simulink model "Fourteen_bus_simscape_V1o1"  (R2026a)
settings: Solver=ode23t  StopTime=12  FixedStep=0.2  RelTol=1e-2  AbsTol=1e-2  EnableMultiTasking=on
libraries: ee_lib x92, nesl_utility x64, fl_lib x25, eeRmsMeasurement x18, slpidlib x5, eeSmGovernor x2, elec_conv_HighZElecRef x1
(part 2 of 3)

== system Fourteen_bus_simscape_V1o1/Bus 7  ==
  Current and Voltage Sensor (Three-Phase) : ee_lib/Sensors & Transducers/Current and Voltage Sensor (Three-Phase)  port_option=ee.enum.threePhasePort.expanded  vMeasurementType=ee.enum.vmeasurement.ll  outputUnit=ee.enum.unit.si  SRated=100000000 V*A  VRated=0.95 V  I_specify=off  I_priority=None  I=[ 0 0 0 ] A  I_nominal_specify=off  I_nominal_value=1  I_nominal_unit=A  V_specify=off  V_priority=None  V=[ 0 0 0 ] V  V_nominal_specify=off  V_nominal_value=1  V_nominal_unit=V
  Demux : Demux  Outputs=3
  PS-Simulink Converter : nesl_utility/PS-Simulink Converter  PhysicalDomain=network_engine_domain  SubClassName=ps_output  LeftPortType=input  RightPortType=output  PseudoPeriodic=off  Frequencies=[]  VectorFormat=1-D array  Unit=1  AffineConversion=off
  PS-Simulink Converter1 : nesl_utility/PS-Simulink Converter  PhysicalDomain=network_engine_domain  SubClassName=ps_output  LeftPortType=input  RightPortType=output  PseudoPeriodic=off  Frequencies=[]  VectorFormat=1-D array  Unit=1  AffineConversion=off
  RMS Measurement : eeRmsMeasurement/RMS Measurement  LabelModeActiveChoice=Total  F=60  SpecifyHarmonics=off  K=[0 1 2]  Ts=0
      settings: LibrarySourceBlock=|
      | ee_sl_lib/Measurements/RMS
      | Measurement
  A : PMIOPort  Side=Left
  B : PMIOPort  Port=2  Side=Left
  C : PMIOPort  Port=3  Side=Left
  a : PMIOPort  Port=4  Side=Right
  b : PMIOPort  Port=5  Side=Right
  c : PMIOPort  Port=6  Side=Right
  Vabc : Outport  VectorParamsAs1DForOutWhenUnconnected=off
  Iabc : Outport  Port=2  VectorParamsAs1DForOutWhenUnconnected=off
  wires:
  PS-Simulink Converter1/1 -> Iabc/1
  Demux/2 -> RMS Measurement/1
  PS-Simulink Converter/1 -> Demux/1
  RMS Measurement/1 -> Vabc/1
  connections:
  Current and Voltage Sensor (Three-Phase)/RConn1 -- PS-Simulink Converter/LConn1
  Current and Voltage Sensor (Three-Phase)/RConn2 -- PS-Simulink Converter1/LConn1
  Current and Voltage Sensor (Three-Phase)/RConn5 -- c/RConn1
  Current and Voltage Sensor (Three-Phase)/RConn4 -- b/RConn1
  Current and Voltage Sensor (Three-Phase)/RConn3 -- a/RConn1
  Current and Voltage Sensor (Three-Phase)/LConn3 -- C/RConn1
  Current and Voltage Sensor (Three-Phase)/LConn1 -- A/RConn1
  Current and Voltage Sensor (Three-Phase)/LConn2 -- B/RConn1

== system Fourteen_bus_simscape_V1o1/Bus 8  ==
  Current and Voltage Sensor (Three-Phase) : ee_lib/Sensors & Transducers/Current and Voltage Sensor (Three-Phase)  port_option=ee.enum.threePhasePort.expanded  vMeasurementType=ee.enum.vmeasurement.ll  outputUnit=ee.enum.unit.si  SRated=100000000 V*A  VRated=1 V  I_specify=off  I_priority=None  I=[ 0 0 0 ] A  I_nominal_specify=off  I_nominal_value=1  I_nominal_unit=A  V_specify=off  V_priority=None  V=[ 0 0 0 ] V  V_nominal_specify=off  V_nominal_value=1  V_nominal_unit=V
  Demux : Demux  Outputs=3
  PS-Simulink Converter : nesl_utility/PS-Simulink Converter  PhysicalDomain=network_engine_domain  SubClassName=ps_output  LeftPortType=input  RightPortType=output  PseudoPeriodic=off  Frequencies=[]  VectorFormat=1-D array  Unit=1  AffineConversion=off
  PS-Simulink Converter1 : nesl_utility/PS-Simulink Converter  PhysicalDomain=network_engine_domain  SubClassName=ps_output  LeftPortType=input  RightPortType=output  PseudoPeriodic=off  Frequencies=[]  VectorFormat=1-D array  Unit=1  AffineConversion=off
  RMS Measurement : eeRmsMeasurement/RMS Measurement  LabelModeActiveChoice=Total  F=60  SpecifyHarmonics=off  K=[0 1 2]  Ts=0
      settings: LibrarySourceBlock=|
      | ee_sl_lib/Measurements/RMS
      | Measurement
  A : PMIOPort  Side=Left
  B : PMIOPort  Port=2  Side=Left
  C : PMIOPort  Port=3  Side=Left
  a : PMIOPort  Port=4  Side=Right
  b : PMIOPort  Port=5  Side=Right
  c : PMIOPort  Port=6  Side=Right
  Vabc : Outport  VectorParamsAs1DForOutWhenUnconnected=off
  Iabc : Outport  Port=2  VectorParamsAs1DForOutWhenUnconnected=off
  wires:
  PS-Simulink Converter1/1 -> Iabc/1
  Demux/2 -> RMS Measurement/1
  PS-Simulink Converter/1 -> Demux/1
  RMS Measurement/1 -> Vabc/1
  connections:
  Current and Voltage Sensor (Three-Phase)/RConn1 -- PS-Simulink Converter/LConn1
  Current and Voltage Sensor (Three-Phase)/RConn2 -- PS-Simulink Converter1/LConn1
  Current and Voltage Sensor (Three-Phase)/RConn5 -- c/RConn1
  Current and Voltage Sensor (Three-Phase)/RConn4 -- b/RConn1
  Current and Voltage Sensor (Three-Phase)/RConn3 -- a/RConn1
  Current and Voltage Sensor (Three-Phase)/LConn3 -- C/RConn1
  Current and Voltage Sensor (Three-Phase)/LConn1 -- A/RConn1
  Current and Voltage Sensor (Three-Phase)/LConn2 -- B/RConn1

== system Fourteen_bus_simscape_V1o1/Bus 9  ==
  Current and Voltage Sensor (Three-Phase) : ee_lib/Sensors & Transducers/Current and Voltage Sensor (Three-Phase)  port_option=ee.enum.threePhasePort.expanded  vMeasurementType=ee.enum.vmeasurement.ll  outputUnit=ee.enum.unit.si  SRated=100000000 V*A  VRated=0.94 V  I_specify=off  I_priority=None  I=[ 0 0 0 ] A  I_nominal_specify=off  I_nominal_value=1  I_nominal_unit=A  V_specify=off  V_priority=None  V=[ 0 0 0 ] V  V_nominal_specify=off  V_nominal_value=1  V_nominal_unit=V
  Demux : Demux  Outputs=3
  PS-Simulink Converter : nesl_utility/PS-Simulink Converter  PhysicalDomain=network_engine_domain  SubClassName=ps_output  LeftPortType=input  RightPortType=output  PseudoPeriodic=off  Frequencies=[]  VectorFormat=1-D array  Unit=1  AffineConversion=off
  PS-Simulink Converter1 : nesl_utility/PS-Simulink Converter  PhysicalDomain=network_engine_domain  SubClassName=ps_output  LeftPortType=input  RightPortType=output  PseudoPeriodic=off  Frequencies=[]  VectorFormat=1-D array  Unit=1  AffineConversion=off
  RMS Measurement : eeRmsMeasurement/RMS Measurement  LabelModeActiveChoice=Total  F=60  SpecifyHarmonics=off  K=[0 1 2]  Ts=0
      settings: LibrarySourceBlock=|
      | ee_sl_lib/Measurements/RMS
      | Measurement
  A : PMIOPort  Side=Left
  B : PMIOPort  Port=2  Side=Left
  C : PMIOPort  Port=3  Side=Left
  a : PMIOPort  Port=4  Side=Right
  b : PMIOPort  Port=5  Side=Right
  c : PMIOPort  Port=6  Side=Right
  Vabc : Outport  VectorParamsAs1DForOutWhenUnconnected=off
  Iabc : Outport  Port=2  VectorParamsAs1DForOutWhenUnconnected=off
  wires:
  PS-Simulink Converter1/1 -> Iabc/1
  Demux/2 -> RMS Measurement/1
  PS-Simulink Converter/1 -> Demux/1
  RMS Measurement/1 -> Vabc/1
  connections:
  Current and Voltage Sensor (Three-Phase)/RConn1 -- PS-Simulink Converter/LConn1
  Current and Voltage Sensor (Three-Phase)/RConn2 -- PS-Simulink Converter1/LConn1
  Current and Voltage Sensor (Three-Phase)/RConn5 -- c/RConn1
  Current and Voltage Sensor (Three-Phase)/RConn4 -- b/RConn1
  Current and Voltage Sensor (Three-Phase)/RConn3 -- a/RConn1
  Current and Voltage Sensor (Three-Phase)/LConn3 -- C/RConn1
  Current and Voltage Sensor (Three-Phase)/LConn1 -- A/RConn1
  Current and Voltage Sensor (Three-Phase)/LConn2 -- B/RConn1

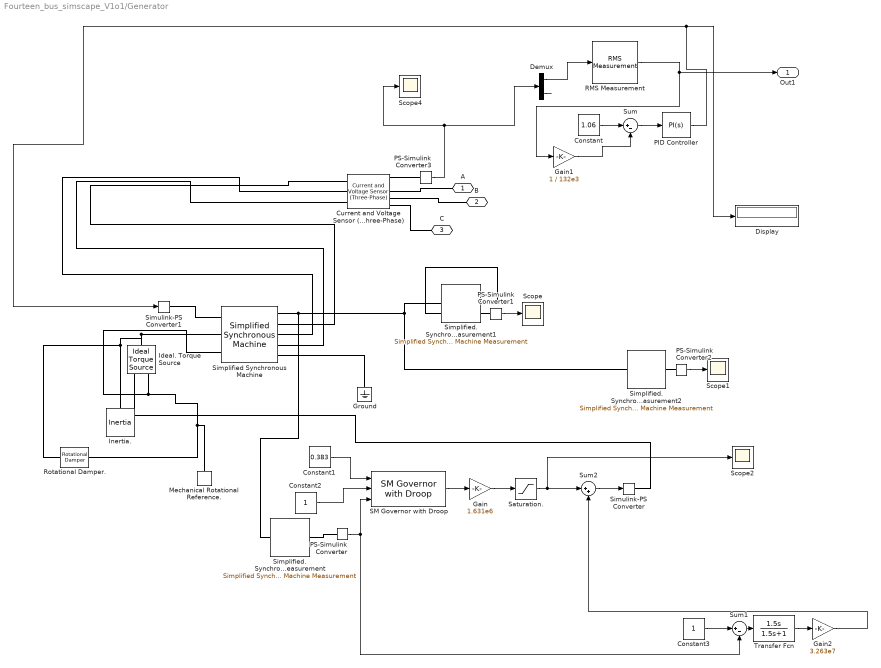
== system Fourteen_bus_simscape_V1o1/Generator ==
  Constant : Constant  Value=1.06
  Constant1 : Constant  Value=0.383
  Constant2 : Constant
  Constant3 : Constant
  Current and Voltage Sensor (Three-Phase) : ee_lib/Sensors & Transducers/Current and Voltage Sensor (Three-Phase)  port_option=ee.enum.threePhasePort.expanded  vMeasurementType=ee.enum.vmeasurement.ll  outputUnit=ee.enum.unit.si  SRated=100000000 V*A  VRated=0.92 V  I_specify=off  I_priority=None  I=[ 0 0 0 ] A  I_nominal_specify=off  I_nominal_value=1  I_nominal_unit=A  V_specify=off  V_priority=None  V=[ 0 0 0 ] V  V_nominal_specify=off  V_nominal_value=1  V_nominal_unit=V
  Demux : Demux  Outputs=3
  Display : Display
  Gain : Gain  Gain=1.631e6
  Gain1 : Gain  Gain=1 / 132e3
  Gain2 : Gain  Gain=3.263e7
  Ground : fl_lib/Electrical/Electrical Elements/Electrical Reference
  Ideal. Torque Source : fl_lib/Mechanical/Mechanical Sources/Ideal Torque Source
  Inertia. : fl_lib/Mechanical/Rotational Elements/Inertia  inertia=3.46e4 kg*m^2  num_ports=foundation.enum.numPorts2.one  w_specify=on  w_priority=High  w=377 rad/s  w_nominal_specify=off  w_nominal_value=1  w_nominal_unit=rad/s  t_specify=off  t_priority=None  t=0 N*m  t_nominal_specify=off  t_nominal_value=1  t_nominal_unit=N*m
  Mechanical Rotational Reference. : fl_lib/Mechanical/Rotational Elements/Mechanical Rotational Reference
  PID Controller : slpidlib/PID Controller  Controller=PI  Form=Parallel  TimeDomain=Continuous-time  UseExternalTs=off  SampleTime=-1  IntegratorMethod=Forward Euler  FilterMethod=Forward Euler  ControllerParametersSource=internal  P=1  I=10  UseKiTs=off  D=0  UseExternalDerivativeSource=off  N=100  UseFilter=on  TunerSelectOption=Transfer Function Based (PID Tuner App)  ZeroCross=off  InitialConditionSource=internal  InitialConditionForIntegrator=1  InitialConditionForFilter=0  DifferentiatorICPrevScaledInput=0  ExternalReset=none  TrackingMode=off  Kt=1  LimitOutput=on  SatLimitsSource=internal  UpperSaturationLimit=1.5  LowerSaturationLimit=0.5  LinearizeAsGain=on  AntiWindupMode=clamping  Kb=1  LimitIntegrator=off  UpperIntegratorSaturationLimit=inf  LowerIntegratorSaturationLimit=-inf  POutMin=[]  POutMax=[]  IOutMin=[]  IOutMax=[]  DOutMin=[]  DOutMax=[]  NOutMin=[]  NOutMax=[]  SumOutMin=[]  SumOutMax=[]  SaturationOutMin=[]  SaturationOutMax=[]  PParamMin=[]  PParamMax=[]  IParamMin=[]  IParamMax=[]  DParamMin=[]  DParamMax=[]  NParamMin=[]  NParamMax=[]  KbParamMin=[]  KbParamMax=[]  KtParamMin=[]  KtParamMax=[]  KbOutMin=[]  KbOutMax=[]  KtOutMin=[]  KtOutMax=[]  IntegratorOutMin=[]  IntegratorOutMax=[]  FilterOutMin=[]  FilterOutMax=[]  SumI1OutMin=[]  SumI1OutMax=[]  SumI2OutMin=[]  SumI2OutMax=[]  SumI3OutMin=[]  SumI3OutMax=[]  SumI4OutMin=[]  SumI4OutMax=[]  SumDOutMin=[]  SumDOutMax=[]  DifferentiatorOutMin=[]  DifferentiatorOutMax=[]  FilterDiffOutCoefMin=[]  FilterDiffOutCoefMax=[]  ReciprocalOutMin=[]  ReciprocalOutMax=[]  SumDenOutMin=[]  SumDenOutMax=[]  SumNumOutMin=[]  SumNumOutMax=[]  DivideOutMin=[]  DivideOutMax=[]  UdiffTsProdOutMin=[]  UdiffTsProdOutMax=[]  NTsProdOutMin=[]  NTsProdOutMax=[]  UintegralTsProdOutMin=[]  UintegralTsProdOutMax=[]  UngainTsProdOutMin=[]  UngainTsProdOutMax=[]  ClampingZeroOutDataTypeStr=Inherit: Inherit via back propagation  ClampingZeroOutMin=[]  ClampingZeroOutMax=[]  FilterDenConstantOutDataTypeStr=Inherit: Inherit via back propagation  FilterDenConstantOutMin=[]  FilterDenConstantOutMax=[]  PCopyOutDataTypeStr=Inherit: Inherit via back propagation  PCopyOutMin=[]  PCopyOutMax=[]  NCopyOutDataTypeStr=Inherit: Inherit via back propagation  NCopyOutMin=[]  NCopyOutMax=[]  IntegratorContinuousStateAttributes=''  IntegratorStateMustResolveToSignalObject=off  IntegratorRTWStateStorageClass=Auto  FilterContinuousStateAttributes=''  FilterStateMustResolveToSignalObject=off  FilterRTWStateStorageClass=Auto  ParallelPVariant=InternalParameters  IdealPVariant=Disabled  IVariant=InternalParameters  DVariant=Disabled  IntegratorVariant=Continuous  SatVariant=Enabled  AWVariant=ContClampingParallel  PCopyVariant=Disabled  TRVariant=Disabled  FdbkBlocksVariant=Forward  IdealPFdbkVariant=Disabled  SatFdbkVariant=Disabled  DerivativeFilterVariant=Disabled  NVariant=Disabled  NCopyVariant=Disabled_SignalSpec  FilterICVariant=Disabled  IntegratorICVariant=InternalICs  ExternalResetVariant=Disabled  TRSumVariant=Passthrough  SumFdbkVariant=Disabled  SumVariant=Sum_PI  TsampFilterVariant=InternalTs  TsampNgainVariant=Passthrough  TsampIntegralVariant=Disabled_SignalSpec  ExternalSaturationOutDataTypeStr=Inherit: Same as second input  DerivativeSourceVariant=Disabled  PreIntVariant=InternalPreInt
  PS-Simulink Converter : nesl_utility/PS-Simulink Converter  PhysicalDomain=network_engine_domain  SubClassName=ps_output  LeftPortType=input  RightPortType=output  PseudoPeriodic=off  Frequencies=[]  VectorFormat=inherit  Unit=inherit  AffineConversion=off
  PS-Simulink Converter1 : nesl_utility/PS-Simulink Converter  PhysicalDomain=network_engine_domain  SubClassName=ps_output  LeftPortType=input  RightPortType=output  PseudoPeriodic=off  Frequencies=[]  VectorFormat=inherit  Unit=inherit  AffineConversion=off
  PS-Simulink Converter2 : nesl_utility/PS-Simulink Converter  PhysicalDomain=network_engine_domain  SubClassName=ps_output  LeftPortType=input  RightPortType=output  PseudoPeriodic=off  Frequencies=[]  VectorFormat=inherit  Unit=inherit  AffineConversion=off
  PS-Simulink Converter3 : nesl_utility/PS-Simulink Converter  PhysicalDomain=network_engine_domain  SubClassName=ps_output  LeftPortType=input  RightPortType=output  PseudoPeriodic=off  Frequencies=[]  VectorFormat=1-D array  Unit=1  AffineConversion=off
  RMS Measurement : eeRmsMeasurement/RMS Measurement  LabelModeActiveChoice=Total  F=60  SpecifyHarmonics=off  K=[0 1 2]  Ts=0
      settings: LibrarySourceBlock=|
      | ee_sl_lib/Measurements/RMS
      | Measurement
  Rotational Damper. : fl_lib/Mechanical/Rotational Elements/Rotational Damper  D=21.6 N*m*s/rad  w_specify=off  w_priority=None  w=0 rad/s  w_nominal_specify=off  w_nominal_value=1  w_nominal_unit=rad/s  t_specify=off  t_priority=None  t=0 N*m  t_nominal_specify=off  t_nominal_value=1  t_nominal_unit=N*m
  SM Governor with Droop : eeSmGovernor/SM Governor with Droop  droop_percentage=5  T_G=0.2  pu_throttle0=.383
      settings: LibrarySourceBlock=|
      | ee_sl_lib/SM Control/SM Governor
      | with Droop
  Saturation. : Saturate  UpperLimit=1.794e6  LowerLimit=0  ZeroCross=off
  Scope{,1..2,4} (4 alike) : Scope
      Scope settings: ActiveDisplayYMinimum=0.99185649896453065  ActiveDisplayYMaximum=1.0031077750720234  DataLoggingVariableName=ScopeData29
      Scope1 settings: ActiveDisplayYMinimum=-0.42563007307096962  ActiveDisplayYMaximum=1.7429831852979154  DataLoggingVariableName=ScopeData30
      Scope2 settings: ActiveDisplayYMinimum=13831.01998574764  ActiveDisplayYMaximum=1.8736373569319628E+6  DataLoggingVariableName=ScopeData31
      Scope4 settings: ActiveDisplayYMinimum=92904.0246764964  ActiveDisplayYMaximum=203246.35987574319
  Simplified Synchronous Machine : ee_lib/Electromechanical/Synchronous/Simplified Synchronous Machine  port_option=ee.enum.threePhasePort.expanded  SRated=615e6 A*V  VRated=132e3 V  FRated=60 Hz  nPolePairs=1  param_unit=ee.enum.unit.pu  R_si=0.0519 Ohm  L_si=8.2589e-04 H  R_pu=0.001  L_pu=0.2995  initialization_option=ee.enum.sm.initialization.steadystate  source_type=ee.enum.sm.load_flow_source_type.Swing  Vmag0=139920 V  Vang0=0 deg  Pt0=232e6 W  Qt0=0 A*V  minimum_pu=0.95  phase_search_range=[-inf, inf] deg  gmin=1e-6 S  connection_option=ee.enum.Connection.wye  angular_position_diff_specify=off  angular_position_diff_priority=None  angular_position_diff=0 rad  angular_position_diff_nominal_specify=off  angular_position_diff_nominal_value=1  angular_position_diff_nominal_unit=rad  pu_psid_specify=off  pu_psid_priority=None  pu_psid=0  pu_psid_nominal_specify=off  pu_psid_nominal_value=1  pu_psid_nominal_unit=1  pu_psiq_specify=off  pu_psiq_priority=None  pu_psiq=0  pu_psiq_nominal_specify=off  pu_psiq_nominal_value=1  pu_psiq_nominal_unit=1  pu_psi0_specify=off  pu_psi0_priority=None  pu_psi0=0  pu_psi0_nominal_specify=off  pu_psi0_nominal_value=1  pu_psi0_nominal_unit=1  angular_torque_specify=off  angular_torque_priority=None  angular_torque=0 N*m  angular_torque_nominal_specify=off  angular_torque_nominal_value=1  angular_torque_nominal_unit=N*m  Tmeas=298.15 K  alpha=3.93e-3 1/K  stator_thermal_mass=100 J/K  rotor_thermal_mass=200 J/K  temperatureA_specify=off  temperatureA_priority=High  temperatureA=25 degC  temperatureA_nominal_specify=off  temperatureA_nominal_value=1  temperatureA_nominal_unit=degC  temperatureB_specify=off  temperatureB_priority=High  temperatureB=25 degC  temperatureB_nominal_specify=off  temperatureB_nominal_value=1  temperatureB_nominal_unit=degC  temperatureC_specify=off  temperatureC_priority=High  temperatureC=25 degC  temperatureC_nominal_specify=off  temperatureC_nominal_value=1  temperatureC_nominal_unit=degC  temperatureR_specify=off  temperatureR_priority=High  temperatureR=25 degC  temperatureR_nominal_specify=off  temperatureR_nominal_value=1  temperatureR_nominal_unit=degC
  Simplified. Synchronous Machine Measurement : ee_lib/Electromechanical/Synchronous/Simplified Synchronous Machine Measurement  output_idx=5
  Simplified. Synchronous Machine Measurement1 : ee_lib/Electromechanical/Synchronous/Simplified Synchronous Machine Measurement  output_idx=5
  Simplified. Synchronous Machine Measurement2 : ee_lib/Electromechanical/Synchronous/Simplified Synchronous Machine Measurement  output_idx=13
  Simulink-PS Converter : nesl_utility/Simulink-PS Converter  PhysicalDomain=network_engine_domain  SubClassName=ps_input  LeftPortType=input  RightPortType=output  PseudoPeriodic=off  Frequencies=[]  NoiseDistribution=none  NoiseParameters=[]  Unit=1  AffineConversion=off  FilteringAndDerivatives=filter  SimscapeFilterOrder=1  InputFilterTimeConstant=0.001  UdotUserProvided=0
  Simulink-PS Converter1 : nesl_utility/Simulink-PS Converter  PhysicalDomain=network_engine_domain  SubClassName=ps_input  LeftPortType=input  RightPortType=output  PseudoPeriodic=off  Frequencies=[]  NoiseDistribution=none  NoiseParameters=[]  Unit=1  AffineConversion=off  FilteringAndDerivatives=filter  SimscapeFilterOrder=1  InputFilterTimeConstant=0.001  UdotUserProvided=0
  Sum : Sum  Inputs=|+-
  Sum1 : Sum  Inputs=|+-
  Sum2 : Sum  Inputs=|++
  Transfer Fcn : TransferFcn  Numerator=[1.5 0]  Denominator=[1.5 1]
  A : PMIOPort  Side=Right
  B : PMIOPort  Port=2  Side=Right
  C : PMIOPort  Port=3  Side=Right
  Out1 : Outport
  wires:
  Gain/1 -> Saturation./1
  Constant1/1 -> SM Governor with Droop/1
  Constant2/1 -> SM Governor with Droop/2
  SM Governor with Droop/1 -> Gain/1
  Saturation./1 -> Sum2/1, Scope2/1
  PS-Simulink Converter1/1 -> Scope/1
  PS-Simulink Converter2/1 -> Scope1/1
  Demux/3 -> ?
  PS-Simulink Converter3/1 -> Demux/1, Scope4/1
  Gain1/1 -> Sum/2
  Sum/1 -> PID Controller/1
  Demux/1 -> RMS Measurement/1
  PID Controller/1 -> Display/1, Simulink-PS Converter1/1
  RMS Measurement/1 -> Out1/1, Gain1/1
  Constant/1 -> Sum/1
  Gain2/1 -> Sum2/2
  Constant3/1 -> Sum1/1
  Sum1/1 -> Transfer Fcn/1
  PS-Simulink Converter/1 -> SM Governor with Droop/3, Sum1/2
  Transfer Fcn/1 -> Gain2/1
  Sum2/1 -> Simulink-PS Converter/1
  connections:
  Rotational Damper./RConn1 -- Mechanical Rotational Reference./LConn1 -- Ideal. Torque Source/RConn2 -- Simplified Synchronous Machine/LConn3
  Simplified. Synchronous Machine Measurement2/LConn1 -- Simplified. Synchronous Machine Measurement1/LConn1 -- Simplified. Synchronous Machine Measurement/LConn1 -- Simplified Synchronous Machine/RConn1
  Simplified Synchronous Machine/RConn5 -- Ground/LConn1
  Rotational Damper./LConn1 -- Inertia./LConn1 -- Ideal. Torque Source/LConn1 -- Simplified Synchronous Machine/LConn2
  Current and Voltage Sensor (Three-Phase)/LConn2 -- Simplified Synchronous Machine/RConn3
  Current and Voltage Sensor (Three-Phase)/LConn3 -- Simplified Synchronous Machine/RConn4
  Simulink-PS Converter/RConn1 -- Ideal. Torque Source/RConn1
  PS-Simulink Converter/LConn1 -- Simplified. Synchronous Machine Measurement/RConn1
  PS-Simulink Converter1/LConn1 -- Simplified. Synchronous Machine Measurement1/RConn1
  PS-Simulink Converter2/LConn1 -- Simplified. Synchronous Machine Measurement2/RConn1
  Current and Voltage Sensor (Three-Phase)/RConn1 -- PS-Simulink Converter3/LConn1
  Current and Voltage Sensor (Three-Phase)/LConn1 -- Simplified Synchronous Machine/RConn2
  Simulink-PS Converter1/RConn1 -- Simplified Synchronous Machine/LConn1
  Current and Voltage Sensor (Three-Phase)/RConn3 -- A/RConn1
  Current and Voltage Sensor (Three-Phase)/RConn5 -- C/RConn1
  Current and Voltage Sensor (Three-Phase)/RConn4 -- B/RConn1

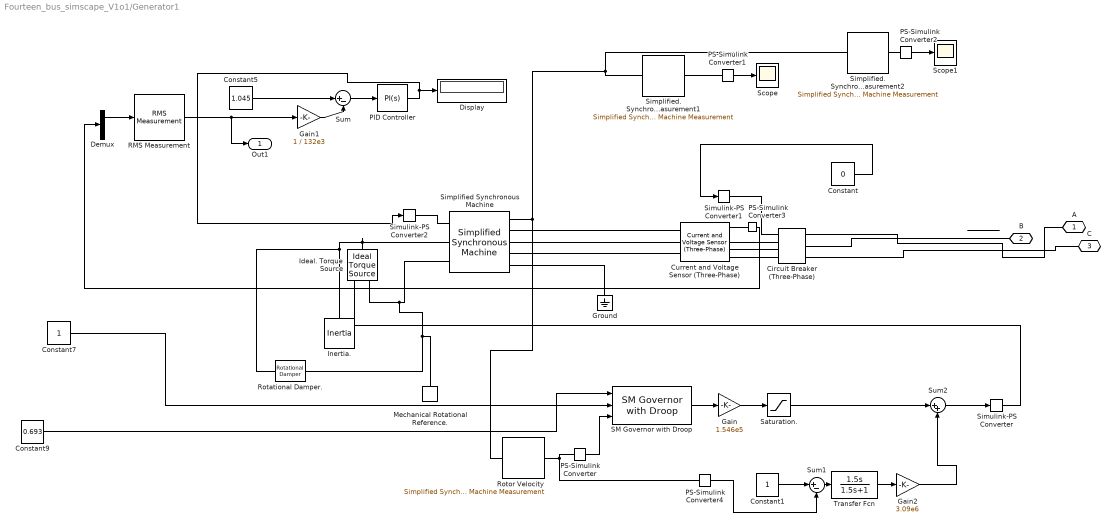
== system Fourteen_bus_simscape_V1o1/Generator1 ==
  Circuit Breaker (Three-Phase) : ee_lib/Switches & Breakers/Circuit Breaker (Three-Phase)  port_option=ee.enum.threePhasePort.expanded  control_port_option=ee.enum.controlport.ps  R_closed=0.001 Ohm  G_open=1e-6 1/Ohm  threshold=0.5 V  breaker_behavior=ee.enum.switches.breakerBehavior.zeroCrossingDisable  i_th=1e-8 A
  Constant : Constant  Value=0
  Constant1 : Constant
  Constant5 : Constant  Value=1.045
  Constant7 : Constant
  Constant9 : Constant  Value=0.693
  Current and Voltage Sensor (Three-Phase) : ee_lib/Sensors & Transducers/Current and Voltage Sensor (Three-Phase)  port_option=ee.enum.threePhasePort.expanded  vMeasurementType=ee.enum.vmeasurement.ll  outputUnit=ee.enum.unit.si  SRated=100000000 V*A  VRated=0.95 V  I_specify=off  I_priority=None  I=[ 0 0 0 ] A  I_nominal_specify=off  I_nominal_value=1  I_nominal_unit=A  V_specify=off  V_priority=None  V=[ 0 0 0 ] V  V_nominal_specify=off  V_nominal_value=1  V_nominal_unit=V
  Demux : Demux  Outputs=3
  Display : Display
  Gain : Gain  Gain=1.546e5
  Gain1 : Gain  Gain=1 / 132e3
  Gain2 : Gain  Gain=3.09e6
  Ground : fl_lib/Electrical/Electrical Elements/Electrical Reference
  Ideal. Torque Source : fl_lib/Mechanical/Mechanical Sources/Ideal Torque Source
  Inertia. : fl_lib/Mechanical/Rotational Elements/Inertia  inertia=3.28e3 kg*m^2  num_ports=foundation.enum.numPorts2.one  w_specify=on  w_priority=High  w=377 rad/s  w_nominal_specify=off  w_nominal_value=1  w_nominal_unit=rad/s  t_specify=off  t_priority=None  t=0 N*m  t_nominal_specify=off  t_nominal_value=1  t_nominal_unit=N*m
  Mechanical Rotational Reference. : fl_lib/Mechanical/Rotational Elements/Mechanical Rotational Reference
  PID Controller : slpidlib/PID Controller  Controller=PI  Form=Parallel  TimeDomain=Continuous-time  UseExternalTs=off  SampleTime=-1  IntegratorMethod=Forward Euler  FilterMethod=Forward Euler  ControllerParametersSource=internal  P=1  I=10  UseKiTs=off  D=0  UseExternalDerivativeSource=off  N=100  UseFilter=on  TunerSelectOption=Transfer Function Based (PID Tuner App)  ZeroCross=off  InitialConditionSource=internal  InitialConditionForIntegrator=1  InitialConditionForFilter=0  DifferentiatorICPrevScaledInput=0  ExternalReset=none  TrackingMode=off  Kt=1  LimitOutput=on  SatLimitsSource=internal  UpperSaturationLimit=1.5  LowerSaturationLimit=0.5  LinearizeAsGain=on  AntiWindupMode=clamping  Kb=1  LimitIntegrator=off  UpperIntegratorSaturationLimit=inf  LowerIntegratorSaturationLimit=-inf  POutMin=[]  POutMax=[]  IOutMin=[]  IOutMax=[]  DOutMin=[]  DOutMax=[]  NOutMin=[]  NOutMax=[]  SumOutMin=[]  SumOutMax=[]  SaturationOutMin=[]  SaturationOutMax=[]  PParamMin=[]  PParamMax=[]  IParamMin=[]  IParamMax=[]  DParamMin=[]  DParamMax=[]  NParamMin=[]  NParamMax=[]  KbParamMin=[]  KbParamMax=[]  KtParamMin=[]  KtParamMax=[]  KbOutMin=[]  KbOutMax=[]  KtOutMin=[]  KtOutMax=[]  IntegratorOutMin=[]  IntegratorOutMax=[]  FilterOutMin=[]  FilterOutMax=[]  SumI1OutMin=[]  SumI1OutMax=[]  SumI2OutMin=[]  SumI2OutMax=[]  SumI3OutMin=[]  SumI3OutMax=[]  SumI4OutMin=[]  SumI4OutMax=[]  SumDOutMin=[]  SumDOutMax=[]  DifferentiatorOutMin=[]  DifferentiatorOutMax=[]  FilterDiffOutCoefMin=[]  FilterDiffOutCoefMax=[]  ReciprocalOutMin=[]  ReciprocalOutMax=[]  SumDenOutMin=[]  SumDenOutMax=[]  SumNumOutMin=[]  SumNumOutMax=[]  DivideOutMin=[]  DivideOutMax=[]  UdiffTsProdOutMin=[]  UdiffTsProdOutMax=[]  NTsProdOutMin=[]  NTsProdOutMax=[]  UintegralTsProdOutMin=[]  UintegralTsProdOutMax=[]  UngainTsProdOutMin=[]  UngainTsProdOutMax=[]  ClampingZeroOutDataTypeStr=Inherit: Inherit via back propagation  ClampingZeroOutMin=[]  ClampingZeroOutMax=[]  FilterDenConstantOutDataTypeStr=Inherit: Inherit via back propagation  FilterDenConstantOutMin=[]  FilterDenConstantOutMax=[]  PCopyOutDataTypeStr=Inherit: Inherit via back propagation  PCopyOutMin=[]  PCopyOutMax=[]  NCopyOutDataTypeStr=Inherit: Inherit via back propagation  NCopyOutMin=[]  NCopyOutMax=[]  IntegratorContinuousStateAttributes=''  IntegratorStateMustResolveToSignalObject=off  IntegratorRTWStateStorageClass=Auto  FilterContinuousStateAttributes=''  FilterStateMustResolveToSignalObject=off  FilterRTWStateStorageClass=Auto  ParallelPVariant=InternalParameters  IdealPVariant=Disabled  IVariant=InternalParameters  DVariant=Disabled  IntegratorVariant=Continuous  SatVariant=Enabled  AWVariant=ContClampingParallel  PCopyVariant=Disabled  TRVariant=Disabled  FdbkBlocksVariant=Forward  IdealPFdbkVariant=Disabled  SatFdbkVariant=Disabled  DerivativeFilterVariant=Disabled  NVariant=Disabled  NCopyVariant=Disabled_SignalSpec  FilterICVariant=Disabled  IntegratorICVariant=InternalICs  ExternalResetVariant=Disabled  TRSumVariant=Passthrough  SumFdbkVariant=Disabled  SumVariant=Sum_PI  TsampFilterVariant=InternalTs  TsampNgainVariant=Passthrough  TsampIntegralVariant=Disabled_SignalSpec  ExternalSaturationOutDataTypeStr=Inherit: Same as second input  DerivativeSourceVariant=Disabled  PreIntVariant=InternalPreInt
  PS-Simulink Converter{,1..4} (5 alike) : nesl_utility/PS-Simulink Converter  PhysicalDomain=network_engine_domain  SubClassName=ps_output  LeftPortType=input  RightPortType=output  PseudoPeriodic=off  Frequencies=[]  VectorFormat=inherit  Unit=inherit  AffineConversion=off
  RMS Measurement : eeRmsMeasurement/RMS Measurement  LabelModeActiveChoice=Total  F=60  SpecifyHarmonics=off  K=[0 1 2]  Ts=0
      settings: LibrarySourceBlock=|
      | ee_sl_lib/Measurements/RMS
      | Measurement
  Rotational Damper. : fl_lib/Mechanical/Rotational Elements/Rotational Damper  D=2.5 N*m*s/rad  w_specify=off  w_priority=None  w=0 rad/s  w_nominal_specify=off  w_nominal_value=1  w_nominal_unit=rad/s  t_specify=off  t_priority=None  t=0 N*m  t_nominal_specify=off  t_nominal_value=1  t_nominal_unit=N*m
  Rotor Velocity : ee_lib/Electromechanical/Synchronous/Simplified Synchronous Machine Measurement  output_idx=5
  SM Governor with Droop : eeSmGovernor/SM Governor with Droop  droop_percentage=5  T_G=0.2  pu_throttle0=0
      settings: LibrarySourceBlock=|
      | ee_sl_lib/SM Control/SM Governor
      | with Droop
  Saturation. : Saturate  UpperLimit=1.70e5  LowerLimit=0  ZeroCross=off
  Scope : Scope
      settings: ActiveDisplayYMinimum=0.94760586598054231  ActiveDisplayYMaximum=1.0354454427456872  DataLoggingVariableName=ScopeData29
  Scope1 : Scope
      settings: ActiveDisplayYMinimum=-5.225588708610692  ActiveDisplayYMaximum=8.40446589134674  DataLoggingVariableName=ScopeData30
  Simplified Synchronous Machine : ee_lib/Electromechanical/Synchronous/Simplified Synchronous Machine  port_option=ee.enum.threePhasePort.expanded  SRated=58.29e6 A*V  VRated=132e3 V  FRated=60 Hz  nPolePairs=1  param_unit=ee.enum.unit.pu  R_si=0.0519 Ohm  L_si=8.2589e-04 H  R_pu=0.001  L_pu=0.2995  initialization_option=ee.enum.sm.initialization.steadystate  source_type=ee.enum.sm.load_flow_source_type.PV  Vmag0=137940 V  Vang0=0 deg  Pt0=40e6 W  Qt0=0 A*V  minimum_pu=0.95  phase_search_range=[-inf, inf] deg  gmin=1e-6 S  connection_option=ee.enum.Connection.wye  angular_position_diff_specify=off  angular_position_diff_priority=None  angular_position_diff=0 rad  angular_position_diff_nominal_specify=off  angular_position_diff_nominal_value=1  angular_position_diff_nominal_unit=rad  pu_psid_specify=off  pu_psid_priority=None  pu_psid=0  pu_psid_nominal_specify=off  pu_psid_nominal_value=1  pu_psid_nominal_unit=1  pu_psiq_specify=off  pu_psiq_priority=None  pu_psiq=0  pu_psiq_nominal_specify=off  pu_psiq_nominal_value=1  pu_psiq_nominal_unit=1  pu_psi0_specify=off  pu_psi0_priority=None  pu_psi0=0  pu_psi0_nominal_specify=off  pu_psi0_nominal_value=1  pu_psi0_nominal_unit=1  angular_torque_specify=off  angular_torque_priority=None  angular_torque=0 N*m  angular_torque_nominal_specify=off  angular_torque_nominal_value=1  angular_torque_nominal_unit=N*m  Tmeas=298.15 K  alpha=3.93e-3 1/K  stator_thermal_mass=100 J/K  rotor_thermal_mass=200 J/K  temperatureA_specify=off  temperatureA_priority=High  temperatureA=25 degC  temperatureA_nominal_specify=off  temperatureA_nominal_value=1  temperatureA_nominal_unit=degC  temperatureB_specify=off  temperatureB_priority=High  temperatureB=25 degC  temperatureB_nominal_specify=off  temperatureB_nominal_value=1  temperatureB_nominal_unit=degC  temperatureC_specify=off  temperatureC_priority=High  temperatureC=25 degC  temperatureC_nominal_specify=off  temperatureC_nominal_value=1  temperatureC_nominal_unit=degC  temperatureR_specify=off  temperatureR_priority=High  temperatureR=25 degC  temperatureR_nominal_specify=off  temperatureR_nominal_value=1  temperatureR_nominal_unit=degC
  Simplified. Synchronous Machine Measurement1 : ee_lib/Electromechanical/Synchronous/Simplified Synchronous Machine Measurement  output_idx=5
  Simplified. Synchronous Machine Measurement2 : ee_lib/Electromechanical/Synchronous/Simplified Synchronous Machine Measurement  output_idx=4
  Simulink-PS Converter : nesl_utility/Simulink-PS Converter  PhysicalDomain=network_engine_domain  SubClassName=ps_input  LeftPortType=input  RightPortType=output  PseudoPeriodic=off  Frequencies=[]  NoiseDistribution=none  NoiseParameters=[]  Unit=1  AffineConversion=off  FilteringAndDerivatives=filter  SimscapeFilterOrder=1  InputFilterTimeConstant=0.001  UdotUserProvided=0
  Simulink-PS Converter1 : nesl_utility/Simulink-PS Converter  PhysicalDomain=network_engine_domain  SubClassName=ps_input  LeftPortType=input  RightPortType=output  PseudoPeriodic=off  Frequencies=[]  NoiseDistribution=none  NoiseParameters=[]  Unit=1  AffineConversion=off  FilteringAndDerivatives=provide  SimscapeFilterOrder=1  InputFilterTimeConstant=0.001  UdotUserProvided=0
  Simulink-PS Converter2 : nesl_utility/Simulink-PS Converter  PhysicalDomain=network_engine_domain  SubClassName=ps_input  LeftPortType=input  RightPortType=output  PseudoPeriodic=off  Frequencies=[]  NoiseDistribution=none  NoiseParameters=[]  Unit=1  AffineConversion=off  FilteringAndDerivatives=filter  SimscapeFilterOrder=1  InputFilterTimeConstant=0.001  UdotUserProvided=0
  Sum : Sum  Inputs=|+-
  Sum1 : Sum  Inputs=|+-
  Sum2 : Sum  Inputs=|++
  Transfer Fcn : TransferFcn  Numerator=[1.5 0]  Denominator=[1.5 1]
  A : PMIOPort  Side=Right
  B : PMIOPort  Port=2  Side=Right
  C : PMIOPort  Port=3  Side=Right
  Out1 : Outport
  wires:
  Gain/1 -> Saturation./1
  Constant9/1 -> SM Governor with Droop/1
  Constant7/1 -> SM Governor with Droop/2
  SM Governor with Droop/1 -> Gain/1
  PS-Simulink Converter/1 -> SM Governor with Droop/3
  PS-Simulink Converter1/1 -> Scope/1
  PS-Simulink Converter2/1 -> Scope1/1
  RMS Measurement/1 -> Out1/1, Gain1/1
  Constant5/1 -> Sum/1
  Gain1/1 -> Sum/2
  Demux/1 -> RMS Measurement/1
  PID Controller/1 -> Simulink-PS Converter2/1, Display/1
  PS-Simulink Converter3/1 -> Demux/1
  Sum/1 -> PID Controller/1
  PS-Simulink Converter4/1 -> Sum1/2
  Sum1/1 -> Transfer Fcn/1
  Transfer Fcn/1 -> Gain2/1
  Constant1/1 -> Sum1/1
  Sum2/1 -> Simulink-PS Converter/1
  Saturation./1 -> Sum2/1
  Gain2/1 -> Sum2/2
  Constant/1 -> Simulink-PS Converter1/1
  connections:
  Rotational Damper./RConn1 -- Mechanical Rotational Reference./LConn1 -- Ideal. Torque Source/RConn2 -- Simplified Synchronous Machine/LConn3
  Simplified. Synchronous Machine Measurement2/LConn1 -- Simplified. Synchronous Machine Measurement1/LConn1 -- Simplified Synchronous Machine/RConn1 -- Rotor Velocity/LConn1
  Simulink-PS Converter2/RConn1 -- Simplified Synchronous Machine/LConn1
  Simplified Synchronous Machine/RConn5 -- Ground/LConn1
  Rotational Damper./LConn1 -- Inertia./LConn1 -- Ideal. Torque Source/LConn1 -- Simplified Synchronous Machine/LConn2
  Simulink-PS Converter/RConn1 -- Ideal. Torque Source/RConn1
  PS-Simulink Converter4/LConn1 -- PS-Simulink Converter/LConn1 -- Rotor Velocity/RConn1
  PS-Simulink Converter1/LConn1 -- Simplified. Synchronous Machine Measurement1/RConn1
  PS-Simulink Converter2/LConn1 -- Simplified. Synchronous Machine Measurement2/RConn1
  Current and Voltage Sensor (Three-Phase)/LConn1 -- Simplified Synchronous Machine/RConn2
  Current and Voltage Sensor (Three-Phase)/LConn2 -- Simplified Synchronous Machine/RConn3
  Current and Voltage Sensor (Three-Phase)/LConn3 -- Simplified Synchronous Machine/RConn4
  Circuit Breaker (Three-Phase)/LConn2 -- Current and Voltage Sensor (Three-Phase)/RConn3
  Circuit Breaker (Three-Phase)/LConn3 -- Current and Voltage Sensor (Three-Phase)/RConn4
  Circuit Breaker (Three-Phase)/LConn4 -- Current and Voltage Sensor (Three-Phase)/RConn5
  Circuit Breaker (Three-Phase)/RConn1 -- A/RConn1
  Circuit Breaker (Three-Phase)/RConn2 -- B/RConn1
  C/RConn1 -- Circuit Breaker (Three-Phase)/RConn3
  PS-Simulink Converter3/LConn1 -- Current and Voltage Sensor (Three-Phase)/RConn1
  ?
  Simulink-PS Converter1/RConn1 -- Circuit Breaker (Three-Phase)/LConn1

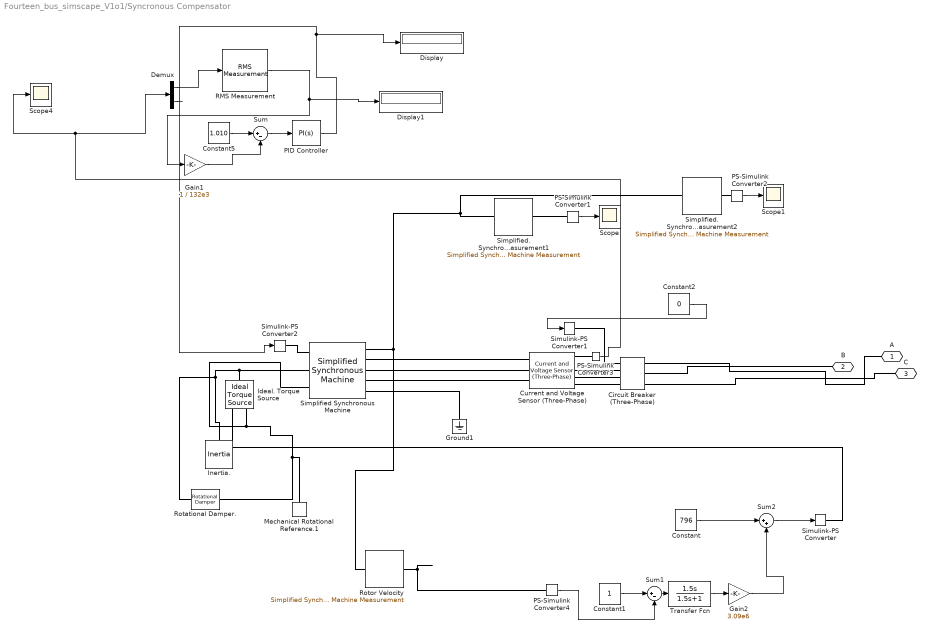
== system Fourteen_bus_simscape_V1o1/Syncronous Compensator ==
  Circuit Breaker (Three-Phase) : ee_lib/Switches & Breakers/Circuit Breaker (Three-Phase)  port_option=ee.enum.threePhasePort.expanded  control_port_option=ee.enum.controlport.ps  R_closed=0.001 Ohm  G_open=1e-6 1/Ohm  threshold=0.5 V  breaker_behavior=ee.enum.switches.breakerBehavior.zeroCrossingDisable  i_th=1e-8 A
  Constant : Constant  Value=796
  Constant1 : Constant
  Constant2 : Constant  Value=0
  Constant5 : Constant  Value=1.010
  Current and Voltage Sensor (Three-Phase) : ee_lib/Sensors & Transducers/Current and Voltage Sensor (Three-Phase)  port_option=ee.enum.threePhasePort.expanded  vMeasurementType=ee.enum.vmeasurement.ll  outputUnit=ee.enum.unit.si  SRated=100000000 V*A  VRated=0.95 V  I_specify=off  I_priority=None  I=[ 0 0 0 ] A  I_nominal_specify=off  I_nominal_value=1  I_nominal_unit=A  V_specify=off  V_priority=None  V=[ 0 0 0 ] V  V_nominal_specify=off  V_nominal_value=1  V_nominal_unit=V
  Demux : Demux  Outputs=3
  Display : Display
  Display1 : Display
  Gain1 : Gain  Gain=1 / 132e3
  Gain2 : Gain  Gain=3.09e6
  Ground1 : fl_lib/Electrical/Electrical Elements/Electrical Reference
  Ideal. Torque Source : fl_lib/Mechanical/Mechanical Sources/Ideal Torque Source
  Inertia. : fl_lib/Mechanical/Rotational Elements/Inertia  inertia=3.4e3 kg*m^2  num_ports=foundation.enum.numPorts2.one  w_specify=on  w_priority=High  w=377 rad/s  w_nominal_specify=off  w_nominal_value=1  w_nominal_unit=rad/s  t_specify=off  t_priority=None  t=0 N*m  t_nominal_specify=off  t_nominal_value=1  t_nominal_unit=N*m
  Mechanical Rotational Reference.1 : fl_lib/Mechanical/Rotational Elements/Mechanical Rotational Reference
  PID Controller : slpidlib/PID Controller  Controller=PI  Form=Parallel  TimeDomain=Continuous-time  UseExternalTs=off  SampleTime=-1  IntegratorMethod=Forward Euler  FilterMethod=Forward Euler  ControllerParametersSource=internal  P=1  I=10  UseKiTs=off  D=0  UseExternalDerivativeSource=off  N=100  UseFilter=on  TunerSelectOption=Transfer Function Based (PID Tuner App)  ZeroCross=off  InitialConditionSource=internal  InitialConditionForIntegrator=1  InitialConditionForFilter=0  DifferentiatorICPrevScaledInput=0  ExternalReset=none  TrackingMode=off  Kt=1  LimitOutput=on  SatLimitsSource=internal  UpperSaturationLimit=1.5  LowerSaturationLimit=0.5  LinearizeAsGain=on  AntiWindupMode=clamping  Kb=1  LimitIntegrator=off  UpperIntegratorSaturationLimit=inf  LowerIntegratorSaturationLimit=-inf  POutMin=[]  POutMax=[]  IOutMin=[]  IOutMax=[]  DOutMin=[]  DOutMax=[]  NOutMin=[]  NOutMax=[]  SumOutMin=[]  SumOutMax=[]  SaturationOutMin=[]  SaturationOutMax=[]  PParamMin=[]  PParamMax=[]  IParamMin=[]  IParamMax=[]  DParamMin=[]  DParamMax=[]  NParamMin=[]  NParamMax=[]  KbParamMin=[]  KbParamMax=[]  KtParamMin=[]  KtParamMax=[]  KbOutMin=[]  KbOutMax=[]  KtOutMin=[]  KtOutMax=[]  IntegratorOutMin=[]  IntegratorOutMax=[]  FilterOutMin=[]  FilterOutMax=[]  SumI1OutMin=[]  SumI1OutMax=[]  SumI2OutMin=[]  SumI2OutMax=[]  SumI3OutMin=[]  SumI3OutMax=[]  SumI4OutMin=[]  SumI4OutMax=[]  SumDOutMin=[]  SumDOutMax=[]  DifferentiatorOutMin=[]  DifferentiatorOutMax=[]  FilterDiffOutCoefMin=[]  FilterDiffOutCoefMax=[]  ReciprocalOutMin=[]  ReciprocalOutMax=[]  SumDenOutMin=[]  SumDenOutMax=[]  SumNumOutMin=[]  SumNumOutMax=[]  DivideOutMin=[]  DivideOutMax=[]  UdiffTsProdOutMin=[]  UdiffTsProdOutMax=[]  NTsProdOutMin=[]  NTsProdOutMax=[]  UintegralTsProdOutMin=[]  UintegralTsProdOutMax=[]  UngainTsProdOutMin=[]  UngainTsProdOutMax=[]  ClampingZeroOutDataTypeStr=Inherit: Inherit via back propagation  ClampingZeroOutMin=[]  ClampingZeroOutMax=[]  FilterDenConstantOutDataTypeStr=Inherit: Inherit via back propagation  FilterDenConstantOutMin=[]  FilterDenConstantOutMax=[]  PCopyOutDataTypeStr=Inherit: Inherit via back propagation  PCopyOutMin=[]  PCopyOutMax=[]  NCopyOutDataTypeStr=Inherit: Inherit via back propagation  NCopyOutMin=[]  NCopyOutMax=[]  IntegratorContinuousStateAttributes=''  IntegratorStateMustResolveToSignalObject=off  IntegratorRTWStateStorageClass=Auto  FilterContinuousStateAttributes=''  FilterStateMustResolveToSignalObject=off  FilterRTWStateStorageClass=Auto  ParallelPVariant=InternalParameters  IdealPVariant=Disabled  IVariant=InternalParameters  DVariant=Disabled  IntegratorVariant=Continuous  SatVariant=Enabled  AWVariant=ContClampingParallel  PCopyVariant=Disabled  TRVariant=Disabled  FdbkBlocksVariant=Forward  IdealPFdbkVariant=Disabled  SatFdbkVariant=Disabled  DerivativeFilterVariant=Disabled  NVariant=Disabled  NCopyVariant=Disabled_SignalSpec  FilterICVariant=Disabled  IntegratorICVariant=InternalICs  ExternalResetVariant=Disabled  TRSumVariant=Passthrough  SumFdbkVariant=Disabled  SumVariant=Sum_PI  TsampFilterVariant=InternalTs  TsampNgainVariant=Passthrough  TsampIntegralVariant=Disabled_SignalSpec  ExternalSaturationOutDataTypeStr=Inherit: Same as second input  DerivativeSourceVariant=Disabled  PreIntVariant=InternalPreInt
  PS-Simulink Converter{1..4} (4 alike) : nesl_utility/PS-Simulink Converter  PhysicalDomain=network_engine_domain  SubClassName=ps_output  LeftPortType=input  RightPortType=output  PseudoPeriodic=off  Frequencies=[]  VectorFormat=inherit  Unit=inherit  AffineConversion=off
  RMS Measurement : eeRmsMeasurement/RMS Measurement  LabelModeActiveChoice=Total  F=60  SpecifyHarmonics=off  K=[0 1 2]  Ts=0
      settings: LibrarySourceBlock=|
      | ee_sl_lib/Measurements/RMS
      | Measurement
  Rotational Damper. : fl_lib/Mechanical/Rotational Elements/Rotational Damper  D=2.1 N*m*s/rad  w_specify=off  w_priority=None  w=0 rad/s  w_nominal_specify=off  w_nominal_value=1  w_nominal_unit=rad/s  t_specify=off  t_priority=None  t=0 N*m  t_nominal_specify=off  t_nominal_value=1  t_nominal_unit=N*m
  Rotor Velocity : ee_lib/Electromechanical/Synchronous/Simplified Synchronous Machine Measurement  output_idx=5
  Scope : Scope
      settings: ActiveDisplayYMinimum=0.98852842414322806  ActiveDisplayYMaximum=1.0076045554902084
  Scope1 : Scope
      settings: ActiveDisplayYMinimum=-7.8389520750323811  ActiveDisplayYMaximum=7.0469005543674257  DataLoggingVariableName=ScopeData9
  Scope4 : Scope
      settings: ActiveDisplayYMinimum=-2.207198407413456E+9  ActiveDisplayYMaximum=1.6372196994728189E+9  DataLoggingVariableName=ScopeData10
  Simplified Synchronous Machine : ee_lib/Electromechanical/Synchronous/Simplified Synchronous Machine  port_option=ee.enum.threePhasePort.expanded  SRated=60e6 A*V  VRated=132e3 V  FRated=60 Hz  nPolePairs=1  param_unit=ee.enum.unit.pu  R_si=0.0519 Ohm  L_si=8.2589e-04 H  R_pu=0.0031  L_pu=0.185  initialization_option=ee.enum.sm.initialization.steadystate  source_type=ee.enum.sm.load_flow_source_type.PV  Vmag0=133320 V  Vang0=0 deg  Pt0=0 W  Qt0=0 A*V  minimum_pu=0.95  phase_search_range=[-inf, inf] deg  gmin=1e-6 S  connection_option=ee.enum.Connection.wye  angular_position_diff_specify=off  angular_position_diff_priority=None  angular_position_diff=0 rad  angular_position_diff_nominal_specify=off  angular_position_diff_nominal_value=1  angular_position_diff_nominal_unit=rad  pu_psid_specify=off  pu_psid_priority=None  pu_psid=0  pu_psid_nominal_specify=off  pu_psid_nominal_value=1  pu_psid_nominal_unit=1  pu_psiq_specify=off  pu_psiq_priority=None  pu_psiq=0  pu_psiq_nominal_specify=off  pu_psiq_nominal_value=1  pu_psiq_nominal_unit=1  pu_psi0_specify=off  pu_psi0_priority=None  pu_psi0=0  pu_psi0_nominal_specify=off  pu_psi0_nominal_value=1  pu_psi0_nominal_unit=1  angular_torque_specify=off  angular_torque_priority=None  angular_torque=0 N*m  angular_torque_nominal_specify=off  angular_torque_nominal_value=1  angular_torque_nominal_unit=N*m  Tmeas=298.15 K  alpha=3.93e-3 1/K  stator_thermal_mass=100 J/K  rotor_thermal_mass=200 J/K  temperatureA_specify=off  temperatureA_priority=High  temperatureA=25 degC  temperatureA_nominal_specify=off  temperatureA_nominal_value=1  temperatureA_nominal_unit=degC  temperatureB_specify=off  temperatureB_priority=High  temperatureB=25 degC  temperatureB_nominal_specify=off  temperatureB_nominal_value=1  temperatureB_nominal_unit=degC  temperatureC_specify=off  temperatureC_priority=High  temperatureC=25 degC  temperatureC_nominal_specify=off  temperatureC_nominal_value=1  temperatureC_nominal_unit=degC  temperatureR_specify=off  temperatureR_priority=High  temperatureR=25 degC  temperatureR_nominal_specify=off  temperatureR_nominal_value=1  temperatureR_nominal_unit=degC
  Simplified. Synchronous Machine Measurement1 : ee_lib/Electromechanical/Synchronous/Simplified Synchronous Machine Measurement  output_idx=5
  Simplified. Synchronous Machine Measurement2 : ee_lib/Electromechanical/Synchronous/Simplified Synchronous Machine Measurement  output_idx=4
  Simulink-PS Converter : nesl_utility/Simulink-PS Converter  PhysicalDomain=network_engine_domain  SubClassName=ps_input  LeftPortType=input  RightPortType=output  PseudoPeriodic=off  Frequencies=[]  NoiseDistribution=none  NoiseParameters=[]  Unit=1  AffineConversion=off  FilteringAndDerivatives=filter  SimscapeFilterOrder=1  InputFilterTimeConstant=0.001  UdotUserProvided=0
  Simulink-PS Converter1 : nesl_utility/Simulink-PS Converter  PhysicalDomain=network_engine_domain  SubClassName=ps_input  LeftPortType=input  RightPortType=output  PseudoPeriodic=off  Frequencies=[]  NoiseDistribution=none  NoiseParameters=[]  Unit=1  AffineConversion=off  FilteringAndDerivatives=provide  SimscapeFilterOrder=1  InputFilterTimeConstant=0.001  UdotUserProvided=0
  Simulink-PS Converter2 : nesl_utility/Simulink-PS Converter  PhysicalDomain=network_engine_domain  SubClassName=ps_input  LeftPortType=input  RightPortType=output  PseudoPeriodic=off  Frequencies=[]  NoiseDistribution=none  NoiseParameters=[]  Unit=1  AffineConversion=off  FilteringAndDerivatives=filter  SimscapeFilterOrder=1  InputFilterTimeConstant=0.001  UdotUserProvided=0
  Sum : Sum  Inputs=|+-
  Sum1 : Sum  Inputs=|+-
  Sum2 : Sum  Inputs=|++
  Transfer Fcn : TransferFcn  Numerator=[1.5 0]  Denominator=[1.5 1]
  A : PMIOPort  Side=Right
  B : PMIOPort  Port=2  Side=Right
  C : PMIOPort  Port=3  Side=Right
  wires:
  Demux/3 -> ?
  PS-Simulink Converter4/1 -> Sum1/2
  Sum/1 -> PID Controller/1
  PS-Simulink Converter1/1 -> Scope/1
  PS-Simulink Converter2/1 -> Scope1/1
  Demux/1 -> RMS Measurement/1
  Transfer Fcn/1 -> Gain2/1
  RMS Measurement/1 -> Display1/1, Gain1/1
  Gain2/1 -> Sum2/2
  PS-Simulink Converter3/1 -> Demux/1, Scope4/1
  Constant5/1 -> Sum/1
  Constant2/1 -> Simulink-PS Converter1/1
  Sum1/1 -> Transfer Fcn/1
  Gain1/1 -> Sum/2
  Sum2/1 -> Simulink-PS Converter/1
  PID Controller/1 -> Display/1, Simulink-PS Converter2/1
  Constant1/1 -> Sum1/1
  Constant/1 -> Sum2/1
  connections:
  Rotational Damper./LConn1 -- Inertia./LConn1 -- Simplified Synchronous Machine/LConn2 -- Ideal. Torque Source/LConn1
  Rotor Velocity/RConn1 -- PS-Simulink Converter4/LConn1
  Rotational Damper./RConn1 -- Mechanical Rotational Reference.1/LConn1 -- Simplified Synchronous Machine/LConn3 -- Ideal. Torque Source/RConn2
  Rotor Velocity/LConn1 -- Simplified Synchronous Machine/RConn1 -- Simplified. Synchronous Machine Measurement2/LConn1 -- Simplified. Synchronous Machine Measurement1/LConn1
  Simulink-PS Converter/RConn1 -- Ideal. Torque Source/RConn1
  Simplified Synchronous Machine/RConn4 -- Current and Voltage Sensor (Three-Phase)/LConn3
  Circuit Breaker (Three-Phase)/RConn2 -- B/RConn1
  PS-Simulink Converter1/LConn1 -- Simplified. Synchronous Machine Measurement1/RConn1
  Simplified Synchronous Machine/LConn1 -- Simulink-PS Converter2/RConn1
  Circuit Breaker (Three-Phase)/LConn3 -- Current and Voltage Sensor (Three-Phase)/RConn4
  PS-Simulink Converter3/LConn1 -- Current and Voltage Sensor (Three-Phase)/RConn1
  Simplified Synchronous Machine/RConn3 -- Current and Voltage Sensor (Three-Phase)/LConn2
  Simulink-PS Converter1/RConn1 -- Circuit Breaker (Three-Phase)/LConn1
  C/RConn1 -- Circuit Breaker (Three-Phase)/RConn3
  Simplified Synchronous Machine/RConn2 -- Current and Voltage Sensor (Three-Phase)/LConn1
  Circuit Breaker (Three-Phase)/RConn1 -- A/RConn1
  Simplified Synchronous Machine/RConn5 -- Ground1/LConn1
  PS-Simulink Converter2/LConn1 -- Simplified. Synchronous Machine Measurement2/RConn1
  Circuit Breaker (Three-Phase)/LConn4 -- Current and Voltage Sensor (Three-Phase)/RConn5
  Circuit Breaker (Three-Phase)/LConn2 -- Current and Voltage Sensor (Three-Phase)/RConn3
